simulink model "fw_imu_tilt"  (R2026b)
settings: Solver=VariableStepAuto
undefined symbols (not defined in the file or in its folder): P, Ts
libraries: simulink x3, mspfiltlib x1
settings Model: Creator=aomar  LastModifiedBy=aomar

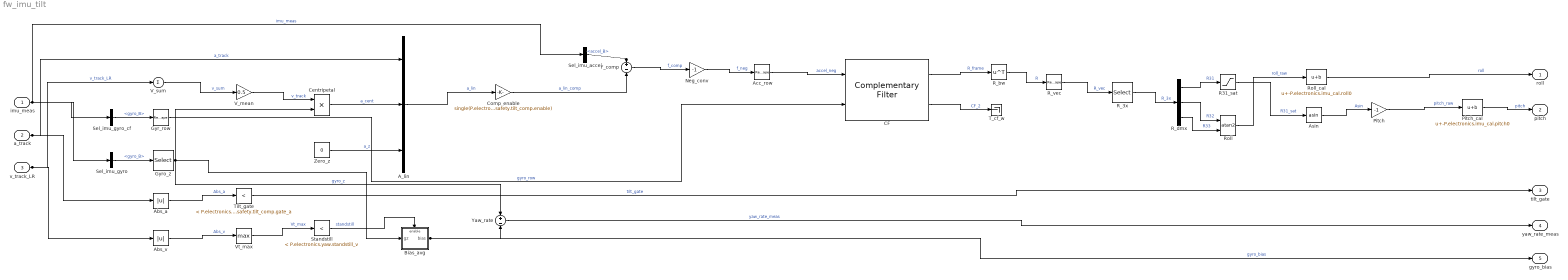
== system fw_imu_tilt ==
  imu_meas : Inport  OutDataTypeStr=Bus: Bus_ImuMeas  SampleTime=Ts.imu
  a_track : Inport  Port=2  OutDataTypeStr=single  SampleTime=Ts.imu
  v_track_LR : Inport  Port=3  OutDataTypeStr=single  PortDimensions=2  SampleTime=Ts.imu
  A_lin : Concatenate  NumInputs=3
  Abs_a : Abs  SaturateOnIntegerOverflow=off
  Abs_v : Abs  SaturateOnIntegerOverflow=off
  Acc_row : Reshape  OutputDimensionality=Customize  OutputDimensions=[1 3]
  Asin : Trigonometry  Operator=asin
  Bias_avg : Subsystem
  CF : mspfiltlib/Complementary Filter  DispRefFrame=ENU  OrientationFormat=Rotation matrix  AccelerometerGain=P.electronics.safety.cf_accel_gain  HasMagnetometer=off  MagnetometerGain=0.01  SimulateUsing=Code generation
  Centripetal : Product
  Comp_enable : Gain  Gain=single(P.electronics.safety.tilt_comp.enable)
  F_comp : Sum  Inputs=+-
  Gyr_row : Reshape  OutputDimensionality=Customize  OutputDimensions=[1 3]
  Gyro_z : Selector  InputPortWidth=3  IndexOptions=Index vector (dialog)  Indices=3  OutputSizes=1
  Neg_conv : Gain  Gain=-1
  Pitch : Gain  Gain=-1
  Pitch_cal : Bias  Bias=-P.electronics.imu_cal.pitch0  SaturateOnIntegerOverflow=off
  R31_sat : Saturate  UpperLimit=1  LowerLimit=-1
  R_3x : Selector  InputPortWidth=9  IndexOptions=Index vector (dialog)  Indices=[3 6 9]  OutputSizes=1
  R_bw : Math  Operator=transpose
  R_dmx : Demux  Outputs=3
  R_vec : Reshape
  Roll : Trigonometry  Operator=atan2
  Roll_cal : Bias  Bias=-P.electronics.imu_cal.roll0  SaturateOnIntegerOverflow=off
  Sel_imu_accel : BusSelector  OutputSignals=accel_B
  Sel_imu_gyro : BusSelector  OutputSignals=gyro_B
  Sel_imu_gyro_cf : BusSelector  OutputSignals=gyro_B
  Standstill : simulink/Logic and Bit Operations/Compare To Constant  relop=<  const=P.electronics.yaw.standstill_v  OutDataTypeStr=boolean
  T_cf_w : Terminator
  Tilt_gate : simulink/Logic and Bit Operations/Compare To Constant  relop=<  const=P.electronics.safety.tilt_comp.gate_a  OutDataTypeStr=boolean
  V_mean : Gain  Gain=0.5
  V_sum : Sum  Inputs=+
  Vt_max : MinMax  Function=max
  Yaw_rate : Sum  Inputs=+-
  Zero_z : Constant  Value=0  OutDataTypeStr=single  SampleTime=-1
  roll : Outport  OutDataTypeStr=single
  pitch : Outport  Port=2  OutDataTypeStr=single
  tilt_gate : Outport  Port=3  OutDataTypeStr=boolean
  yaw_rate_meas : Outport  Port=4  OutDataTypeStr=single
  gyro_bias : Outport  Port=5  OutDataTypeStr=single
  wires:
  imu_meas/1 -> Sel_imu_gyro/1, Sel_imu_accel/1, Sel_imu_gyro_cf/1  "imu_meas"
  a_track/1 -> A_lin/1, Abs_a/1  "a_track"
  v_track_LR/1 -> V_sum/1, Abs_v/1  "v_track_LR"
  Sel_imu_gyro_cf/1 -> Gyr_row/1  "<gyro_B>"
  Sel_imu_gyro/1 -> Gyro_z/1  "<gyro_B>"
  V_sum/1 -> V_mean/1  "v_sum"
  Gyr_row/1 -> CF/2  "gyro_row"
  Abs_a/1 -> Tilt_gate/1  "Abs_a"
  Abs_v/1 -> Vt_max/1  "Abs_v"
  Gyro_z/1 -> Bias_avg/1(gz), Yaw_rate/1, Centripetal/2  "gyro_z"
  V_mean/1 -> Centripetal/1  "v_track"
  Tilt_gate/1 -> tilt_gate/1  "tilt_gate"
  Vt_max/1 -> Standstill/1  "Vt_max"
  Centripetal/1 -> A_lin/2  "a_cent"
  Zero_z/1 -> A_lin/3  "a_z"
  Standstill/1 -> Bias_avg/Enable  "standstill"
  A_lin/1 -> Comp_enable/1  "a_lin"
  Bias_avg/1(bias) -> gyro_bias/1, Yaw_rate/2  "gyro_bias"
  Yaw_rate/1 -> yaw_rate_meas/1  "yaw_rate_meas"
  Comp_enable/1 -> F_comp/2  "a_lin_comp"
  Sel_imu_accel/1 -> F_comp/1  "<accel_B>"
  F_comp/1 -> Neg_conv/1  "f_comp"
  Neg_conv/1 -> Acc_row/1  "f_neg"
  Acc_row/1 -> CF/1  "accel_neg"
  CF/1 -> R_bw/1  "R_frame"
  CF/2 -> T_cf_w/1  "CF_2"
  R_bw/1 -> R_vec/1  "R"
  R_vec/1 -> R_3x/1  "R_vec"
  R_3x/1 -> R_dmx/1  "R_3x"
  R_dmx/1 -> R31_sat/1  "R31"
  R_dmx/2 -> Roll/1  "R32"
  R_dmx/3 -> Roll/2  "R33"
  R31_sat/1 -> Asin/1  "R31_sat"
  Roll/1 -> Roll_cal/1  "roll_raw"
  Asin/1 -> Pitch/1  "Asin"
  Roll_cal/1 -> roll/1  "roll"
  Pitch/1 -> Pitch_cal/1  "pitch_raw"
  Pitch_cal/1 -> pitch/1  "pitch"

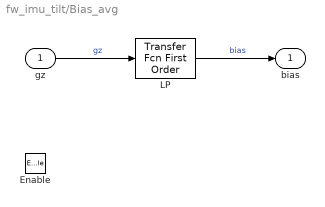
== system fw_imu_tilt/Bias_avg ==
  gz : Inport
  Enable : EnablePort
  LP : simulink/Discrete/Transfer Fcn First Order  PoleZ=exp(-Ts.imu/P.electronics.yaw.tau_bias)  ICPrevOutput=0  DoSatur=off
  bias : Outport  InitialOutput=single(0)
  wires:
  gz/1 -> LP/1  "gz"
  LP/1 -> bias/1  "bias"
